simulink model "test_SimulinkMdl3LPV_IPCa"  (R2019b)
settings: Solver=FixedStepAuto  StartTime=0.0  StopTime=400  FixedStep=DT  RelTol=1e-3
values from neighbouring files (symbols this model uses):
  DT = 0.008    [dataDLR.m]    (also in generateReport.m; initLPVParam.m; initWorkspace.m; runCalculateEvalCriteria.m)
  Lin_points : value not decoded    [DD_test.sldd]
  OutList = OutTable.Properties.VariableNames    [initLPVParam.m]    (also in testCtrl.m; testOutList.m = cell(40, 1); testqLPV.m = cell(40, 1))
  wecs = 3.0    [DD_test.sldd]    (also in dataDLR.m = struct; testOutList.m = struct; testqLPV.m = struct)
undefined symbols (not defined in the file or in its folder): Rotor_Lambda, strmatch, sys12d_w
libraries: cstblocks x1
settings Model: DataDictionary=DD_test.sldd  ExtModeTrigMode=oneshot  ExtModeArmWhenConnect=off  Creator=Hazim Namik  LastModifiedBy=ditt_aj
settings DataIOCC: LimitDataPoints=on  SaveFormat=Array  ReturnWorkspaceOutputs=off
settings OptimizationCC: BlockReduction=off  BooleanDataType=off  LifeSpan=inf
settings DebuggingCC: SaveWithParameterizedLinksMsg=none  UnderspecifiedInitializationDetection=Classic  MergeDetectMultiDrivingBlocksExec=none  SignalResolutionControl=TryResolveAllWithWarning  SFUnexpectedBacktrackingDiag=warning  SFNoUnconditionalDefaultTransitionDiag=warning  SFExecutionAtInitializationDiag=none  ArithmeticOperatorsInVariantConditions=warning
settings HardwareCC: ProdBitPerPointer=32  ProdBitPerSizeT=32  ProdBitPerPtrDiffT=32  ProdLargestAtomicFloat=None  ProdIntDivRoundTo=Undefined  ProdEndianess=Unspecified  ProdWordSize=32  ProdHWDeviceType=32-bit Generic  TargetUnknown=on
settings ModelReferenceCC: PropagateSignalLabelsOutOfModel=off
settings SFSimCC: SimUseLocalCustomCode=off  CustomCodeUndefinedFunction=UseInterfaceOnly
settings RTWCC: RTWUseLocalCustomCode=off
settings CodeAppCC: StateflowObjectComments=on
settings GRTTargetCC: TargetLangStandard=C89/C90 (ANSI)  GeneratePreprocessorConditionals=Disable all
settings ConfigComp: CovMetricSettings=dw  CovHtmlReporting=on  CovSaveCumulativeToWorkspaceVar=on  CovSaveSingleToWorkspaceVar=on  CovExternalEMLEnable=off

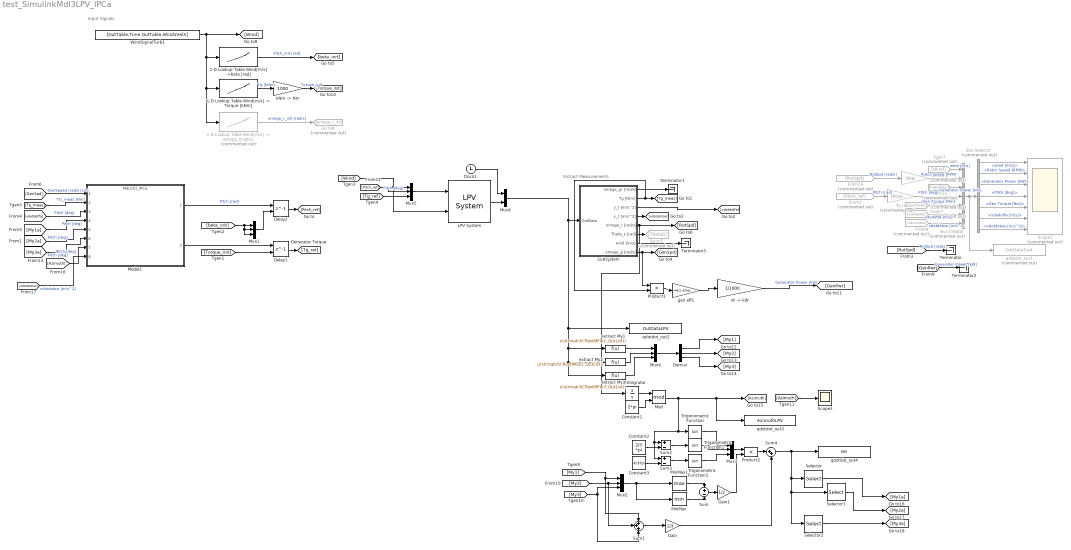
== system test_SimulinkMdl3LPV_IPCa ==
  note: Extract Measurements
  note: Input Signals
  "1-D Lookup Table Wind[m/s] -> Torque [kNm]" : Lookup_n-D  NumberOfTableDimensions=1  BreakpointsForDimension1=Lin_points.V  BreakpointsForDimension2=Rotor_Lambda  Table=Lin_points.Torque  InternalRulePriority=Speed  RndMeth=Simplest  InputSameDT=on
  "1-D Lookup Table Wind[m/s] -> omega_r[rad/s]" : Lookup_n-D  Commented=on  NumberOfTableDimensions=1  BreakpointsForDimension1=Lin_points.V  BreakpointsForDimension2=Rotor_Lambda  Table=Lin_points.RSpeed  InternalRulePriority=Speed  RndMeth=Simplest  InputSameDT=on
  1-D Lookup Table Wind[m/s] ->beta [rad] : Lookup_n-D  NumberOfTableDimensions=1  BreakpointsForDimension1=Lin_points.V  BreakpointsForDimension2=Rotor_Lambda  Table=Lin_points.Pitch  InternalRulePriority=Speed  RndMeth=Simplest  InputSameDT=on
  Bus Creator : BusCreator  Commented=on  Inputs=7
  Bus Selector : BusSelector  Commented=on  OutputSignals=wind [m/s],Rotor Speed [RPM],Generator Power [kW],Pitch [deg],Gen Torque [Nm],xdodotfa [m/s],xdotdotsw [m/s^2]
  Clock1 : Clock
  Constant1 : Constant  Value=2*pi
  Constant2 : Constant  Value=2/3 *pi
  Constant3 : Constant  Value=4/3*pi
  Delay1 : Delay  DelayLength=1  InitialConditionSource=Input port
      settings: InputPortMap=u0,p4
  Delay2 : Delay  DelayLength=1  InitialConditionSource=Input port
      settings: InputPortMap=u0,p4
  Demux : Demux  Outputs=3
  From14 : From  Commented=on  GotoTag=RotSpd
      settings: CloseFcn=tagdialog Close
  From15 : From  Commented=on  GotoTag=GenPwr
      settings: CloseFcn=tagdialog Close
  From2 : From  Commented=on  GotoTag=Pitch_ref
      settings: CloseFcn=tagdialog Close
  From7 : From  Commented=on  GotoTag=xdotdotfa
      settings: CloseFcn=tagdialog Close
  From8 : From  Commented=on  GotoTag=xdotdotsw
      settings: CloseFcn=tagdialog Close
  Gain : Gain  Gain=1/3
  Gain1 : Gain  Gain=1/2
  Go to7 : Goto  Commented=on  GotoTag=ThetaS
  Go to8 : Goto  Commented=on  GotoTag=omega_r_init
  Integrator : Integrator
  LPV System : cstblocks/Linear Parameter Varying/LPV System  sys=sysd  x0=x0  uOffset=uoff  yOffset=yoff  xOffset=xoff  opEquilOption=on  dxOffset=0  sysFixedOption=Use the first model in state-space array  sysFixed=sys12d_w(:,:,4)  AFixed=false  BFixed=false  CFixed=false  DFixed=false  uDelayFixed=false  yDelayFixed=false  iDelayFixed=false  IMethod=Nearest  EMethod=Clip  IndexSearch=Binary search  IndexBegin=on  OutputX=off  OutputXdot=off  OutputLTI=off  OutputOP=off  DataType=double  SimMode=Interpreted execution  InitBufferSize=1024  FixedBuffer=off
      settings: SourceProductName=Control System Toolbox  SourceProductBaseCode=CT
  MinMax : MinMax
  MinMax1 : MinMax  Function=max
  Mod : Math  Operator=mod  SaturateOnIntegerOverflow=on
  Model1 : ModelReference  ModelNameDialog=MdLCtrl_IPCa.slx  SimulationMode=Normal  ModelReferenceVersion=1.34
  Mux{1..5} (5 alike) : Mux  Inputs=3
  Mux6 : Mux  Inputs=2
  Product1 : Product  RndMeth=Zero
  Product2 : Product  RndMeth=Zero
  Scope1 : Scope  Commented=on  NumInputPorts=7
      settings: Tag=Scope
  Scope3 : Scope
  Selector : Selector  InputPortWidth=3  IndexOptions=Index vector (dialog)  Indices=1  OutputSizes=1
  Selector1 : Selector  InputPortWidth=3  IndexOptions=Index vector (dialog)  Indices=2  OutputSizes=1
  Selector2 : Selector  InputPortWidth=3  IndexOptions=Index vector (dialog)  Indices=3  OutputSizes=1
  Subsystem : Subsystem
  Sum : Sum  Inputs=+-
  Sum1 : Sum  Inputs=+++
  Sum2 : Sum  Inputs=+-
  Sum3 : Sum  Inputs=+-
  Sum4 : Sum  Inputs=|++
  Terminator{,1..3} (4 alike) : Terminator
  Tgen6 : From  Commented=on  GotoTag=Tg_meas
      settings: CloseFcn=tagdialog Close
  Tgen7 : From  Commented=on  GotoTag=Wind
      settings: CloseFcn=tagdialog Close
  To rad/s2 : Gain  Commented=on  Gain=30/pi
  To rad/s3 : Gain  Commented=on  Gain=180/pi
  Trigonometric Function : Trigonometry
  Trigonometric Function1 : Trigonometry
  Trigonometric Function2 : Trigonometry
  "W -> kW" : Gain  Gain=1/1000
  WindSignalTurb1 : FromWorkspace  VariableName=[OutTable.Time OutTable.Wind1VelX]  SampleTime=DT  OutputAfterFinalValue=Holding final value
  extract My1 : Fcn  Expr=u(strmatch('RootMFlp1',OutList))
  extract My2 : Fcn  Expr=u(strmatch('RootMFlp2',OutList))
  extract My3 : Fcn  Expr=u(strmatch('RootMFlp3',OutList))
  gen eff1 : Gain  Gain=wecs.etag
  "kNm -> Nm" : Gain  Gain=1000
  qdotdot_out1 : ToWorkspace  Commented=on  VariableName=OutDataTest  SampleTime=-1
  qdotdot_out2 : ToWorkspace  VariableName=OutDataLPV  SampleTime=-1
  qdotdot_out3 : ToWorkspace  VariableName=AzimuthLPV  SampleTime=-1
  qdotdot_out4 : ToWorkspace  VariableName=MY  SampleTime=-1
  wires:
  [Tg_meas] -> Model1/2  "TG_meas [Nm]"
  [xdotdotfa] -> Model1/3  "Pitch [deg]"
  [My1a] -> Model1/4  "Pitch [deg]"
  [GenSpd] -> Model1/1  "GenSpeed [rad/s] LSS"
  Subsystem/1(omega_gr [rad/s]) -> Terminator1/1
  Subsystem/8(omega_g [rad/s]) -> [GenSpd], Product1/1
  Subsystem/3(y_t [m/s^2]) -> [xdotdotfa]
  Subsystem/6(Theta_s [rad]) -> Go to7/1
  Bus Selector/3 -> Scope1/3  "<Generator Power [kW]>"
  Bus Selector/7 -> Scope1/7  "<xdotdotsw [m/s^2]>"
  To rad/s2/1 -> Bus Creator/2  "Rotor Speed [RPM]"
  From15/1 -> Bus Creator/3  "Generator Power [kW]"
  Tgen6/1 -> Bus Creator/5  "Gen Torque [Nm]"
  From8/1 -> Bus Creator/7  "xdotdotsw [m/s^2]"
  Bus Creator/1 -> Bus Selector/1, qdotdot_out1/1
  Bus Selector/6 -> Scope1/6  "<xdodotfa [m/s]>"
  To rad/s3/1 -> Bus Creator/4  "Pitch [deg]"
  Tgen7/1 -> Bus Creator/1  "wind [m/s]"
  Bus Selector/4 -> Scope1/4  "<Pitch [deg]>"
  From2/1 -> To rad/s3/1  "Pitch [rad]"
  From7/1 -> Bus Creator/6  "xdodotfa [m/s]"
  From14/1 -> To rad/s2/1  "RotSpd [rad/s]"
  Bus Selector/2 -> Scope1/2  "<Rotor Speed [RPM]>"
  Bus Selector/5 -> Scope1/5  "<Gen Torque [Nm]>"
  Bus Selector/1 -> Scope1/1  "<wind [m/s]>"
  Mux6/1 -> extract My3/1, extract My2/1, extract My1/1, qdotdot_out2/1, Subsystem/1(OutData)
  "W -> kW"/1 -> [GenPwr]  "Generator Power [kW]"
  gen eff1/1 -> "W -> kW"/1
  Product1/1 -> gen eff1/1
  Subsystem/4(x_t [m/s^2]) -> [xdotdotsw]
  Subsystem/7(wind [m/s]) -> Terminator3/1
  [My3] -> Sum1/3, Mux2/3
  [My1] -> Sum1/1, Mux2/1
  [My2] -> Mux2/2, Sum1/2
  Mux2/1 -> MinMax1/1, MinMax/1
  [Azimuth] -> Scope3/1
  Integrator/1 -> Mod/1
  Constant1/1 -> Mod/2
  Subsystem/5(omega_r [rad/s]) -> [RotSpd], Integrator/1
  Mod/1 -> Sum3/1, Sum2/1, Trigonometric Function/1, qdotdot_out3/1, [Azimuth]
  MinMax1/1 -> Sum/1
  MinMax/1 -> Sum/2
  Sum/1 -> Gain1/1
  Sum1/1 -> Gain/1
  Trigonometric Function/1 -> Mux3/1
  Constant2/1 -> Sum2/2
  Constant3/1 -> Sum3/2
  Sum2/1 -> Trigonometric Function1/1
  Sum3/1 -> Trigonometric Function2/1
  Gain1/1 -> Product2/2
  Trigonometric Function1/1 -> Mux3/2
  Trigonometric Function2/1 -> Mux3/3
  Mux3/1 -> Product2/1
  Product2/1 -> Sum4/1
  Sum4/1 -> Selector2/1, Selector1/1, Selector/1, qdotdot_out4/1
  extract My1/1 -> Mux4/1
  extract My2/1 -> Mux4/2
  extract My3/1 -> Mux4/3
  [My2a] -> Model1/5  "Pitch [deg]"
  [My3a] -> Model1/6  "Pitch [deg]"
  [Azimuth] -> Model1/7  "Pitch [deg]"
  [xdotdotsw] -> Model1/8  "xdotdotsw [m/s^2]"
  Demux/3 -> [My3]
  Demux/1 -> [My1]
  Demux/2 -> [My2]
  Mux4/1 -> Demux/1
  [Wind] -> LPV System/2, Mux5/1
  [Tg_ref] -> Mux5/3
  LPV System/1 -> Mux6/2
  [Pitch_ref] -> Mux5/2  "Pitch [deg]"
  Mux5/1 -> LPV System/1
  Clock1/1 -> Mux6/1
  Model1/2 -> Delay1/1
  Delay1/1 -> [Tg_ref]
  "kNm -> Nm"/1 -> [Torque_init]  "Torque_init"
  WindSignalTurb1/1 -> [Wind], "1-D Lookup Table Wind[m/s] -> omega_r[rad/s]"/1, "1-D Lookup Table Wind[m/s] -> Torque [kNm]"/1, 1-D Lookup Table Wind[m/s] ->beta [rad]/1
  1-D Lookup Table Wind[m/s] ->beta [rad]/1 -> [beta_init]  "Pitch_init [rad]"
  "1-D Lookup Table Wind[m/s] -> Torque [kNm]"/1 -> "kNm -> Nm"/1  "Tg [kNm]"
  "1-D Lookup Table Wind[m/s] -> omega_r[rad/s]"/1 -> Go to8/1  "omega_r_init [rad/s]"
  [Torque_init] -> Delay1/2
  Delay2/1 -> [Pitch_ref]
  Model1/1 -> Delay2/1  "Pitch [rad]"
  Mux1/1 -> Delay2/2
  [beta_init] -> Mux1/3, Mux1/2, Mux1/1
  Subsystem/2(Tg [N/m]) -> [Tg_meas], Product1/2
  [RotSpd] -> Terminator/1  "RotSpd [rad/s]"
  [GenPwr] -> Terminator2/1  "Generator Power [kW]"
  Selector1/1 -> [My2a]
  Selector/1 -> [My1a]
  Selector2/1 -> [My3a]
  Gain/1 -> Sum4/2

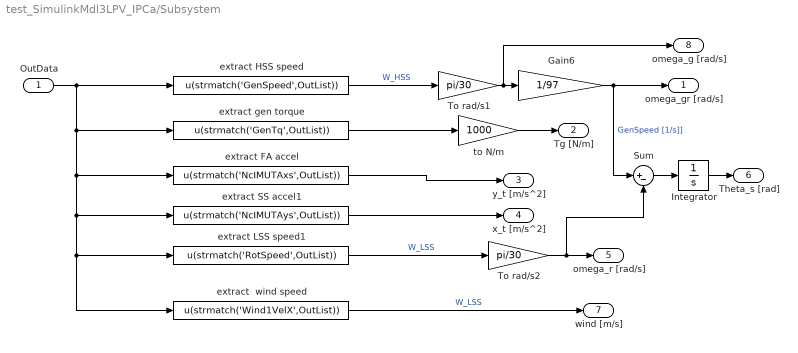
== system test_SimulinkMdl3LPV_IPCa/Subsystem ==
  OutData : Inport
  Gain6 : Gain  Gain=1/97
  Integrator : Integrator
  Sum : Sum  Inputs=|+-
  To rad/s1 : Gain  Gain=pi/30
  To rad/s2 : Gain  Gain=pi/30
  extract  wind speed : Fcn  Expr=u(strmatch('Wind1VelX',OutList))
  extract FA accel : Fcn  Expr=u(strmatch('NcIMUTAxs',OutList))
  extract HSS speed : Fcn  Expr=u(strmatch('GenSpeed',OutList))
  extract LSS speed1 : Fcn  Expr=u(strmatch('RotSpeed',OutList))
  extract SS accel1 : Fcn  Expr=u(strmatch('NcIMUTAys',OutList))
  extract gen torque : Fcn  Expr=u(strmatch('GenTq',OutList))
  to N/m : Gain  Gain=1000
  omega_gr [rad/s] : Outport  VectorParamsAs1DForOutWhenUnconnected=off
  Tg [N/m] : Outport  Port=2  VectorParamsAs1DForOutWhenUnconnected=off
  y_t [m/s^2] : Outport  Port=3  VectorParamsAs1DForOutWhenUnconnected=off
  x_t [m/s^2] : Outport  Port=4  VectorParamsAs1DForOutWhenUnconnected=off
  omega_r [rad/s] : Outport  Port=5  VectorParamsAs1DForOutWhenUnconnected=off
  Theta_s [rad] : Outport  Port=6  VectorParamsAs1DForOutWhenUnconnected=off
  wind [m/s] : Outport  Port=7  VectorParamsAs1DForOutWhenUnconnected=off
  omega_g [rad/s] : Outport  Port=8  VectorParamsAs1DForOutWhenUnconnected=off
  wires:
  to N/m/1 -> Tg [N/m]/1
  OutData/1 -> extract HSS speed/1, extract gen torque/1, extract  wind speed/1, extract LSS speed1/1, extract SS accel1/1, extract FA accel/1
  extract FA accel/1 -> y_t [m/s^2]/1
  extract HSS speed/1 -> To rad/s1/1  "W_HSS"
  extract gen torque/1 -> to N/m/1
  extract SS accel1/1 -> x_t [m/s^2]/1
  To rad/s1/1 -> omega_g [rad/s]/1, Gain6/1
  extract LSS speed1/1 -> To rad/s2/1  "W_LSS"
  Gain6/1 -> omega_gr [rad/s]/1, Sum/1  "GenSpeed [1/s]]"
  To rad/s2/1 -> Sum/2, omega_r [rad/s]/1
  Sum/1 -> Integrator/1
  Integrator/1 -> Theta_s [rad]/1
  extract  wind speed/1 -> wind [m/s]/1  "W_LSS"
